simulink model "Palak_Plant_V1"  (R2025a)
settings: Solver=VariableStepAuto  StartTime=0.0  StopTime=10.0  RelTol=1e-3
settings Model: Creator=palak  LastModifiedBy=palak

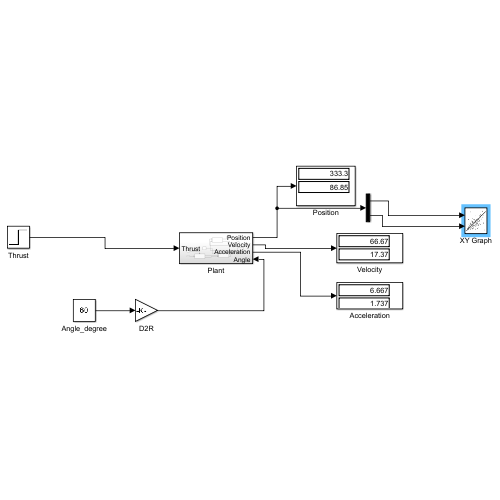
[thumbnail: Simulink's stored preview of the top-level diagram]
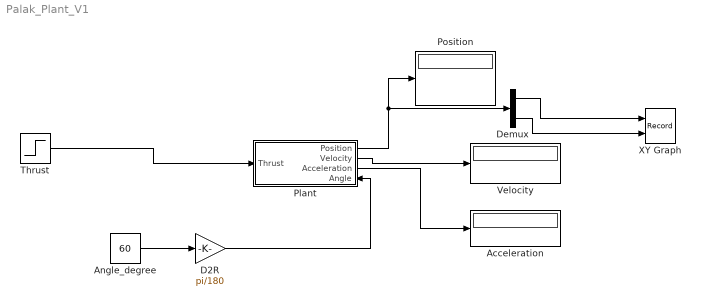
== system Palak_Plant_V1 ==
  Acceleration : Display
  Angle_degree : Constant  Value=60
  D2R : Gain  Gain=pi/180
  Demux : Demux  Outputs=2
  Plant : Subsystem
      settings: PortSchema="{\"entries\":[{\"content\":{\"sides\":[{\"content\":{\"connectorIds\":[\"In1\"]},\"type\":\"ConnectorPlacement.EquallySpacedRectSide\",\"uuid\":\"5de75d20-e3de-4891-9f30-3a0def6c848b\"},{\"content\":{\"connectorIds\":[\"Out1\",\"Out2\",\"Out3\",\"In2\"],\"side\":\"RIGHT\"},\"type\":\"ConnectorPlacement.EquallySpacedRectSide\",\"uuid\":\"db51dd8a-e2b5-4d79-9796-924119c6ed6f\"},{\"content\":{\"side\":\"TOP\"},\"type\":\"ConnectorPlacement.EquallySpacedRectSide\",\"uuid\":\"19ab0691-ef15-4f63-9283-6db2c82ddebe\"}]},\"type\":\"ConnectorPlacement.EquallySpacedConnector\",\"uuid\":\"28e9291f-ce5a-4baf-96c8-583588e41189\"}],\"packageUris\":[\"http://schema.mathworks.com/mf0/Connector/R2020b\"],\"version\":\"1.0\"}"
  Position : Display
  Thrust : Step  Time=0  After=200  SampleTime=0
  Velocity : Display
  XY Graph : Record  NumPorts=2.0  FileSettingsInternal="{\"entries\":[{\"content\":{\"excelSettings\":{\"content\":{},\"type\":\"Streamout.ExcelSettings\"},\"parquetSettings\":{\"content\":{},\"type\":\"Streamout.ParquetSettings\"}},\"type\":\"Streamout.FileSettingStorage\",\"uuid\":\"\"}],\"packageUris\":[\"http:\\/\\/schema.mathworks.com\\/mf0\\/streamout_blocks\\/R2020a\"],\"version\":\"1.0\"}"  FrameSettings=[0, 0]  Layout=[1 1]  SignalsInternal="{\"entries\":[{\"content\":{\"signals\":[{\"content\":{\"blockPath\":[],\"dimensions\":[1],\"domain\":\"\",\"lineColor\":\"#0072bd\",\"lineWidth\":2,\"plots\":[ 1 ],\"port\":1,\"sid\":[\"\"],\"signalID\":1,\"signalName\":\"Demux:1\"},\"type\":\"RecordBlkView.Signal\",\"uuid\":\"\"},{\"content\":{\"blockPath\":[],\"dimensions\":[1],\"domain\":\"\",\"lineColor\":\"#d95319\",\"lineWidth\":2,\"plots\":[ 1 ],\"port\":2,\"sid\":[\"\"],\"signalID\":2,\"signalName\":\"Demux:2\"},\"type\":\"RecordBlkView.Signal\",\"uuid\":\"\"}]},\"type\":\"RecordBlkView.InputSignals\",\"uuid\":\"\"}],\"packageUris\":[\"http:\\/\\/schema.mathworks.com\\/mf0\\/streamout_blocks\\/R2020a\"],\"version\":\"1.0\"}"  VisualizationBindings="{\"xyplotplugin\":{\"info\":[{\"series\":[{\"bindingParametersList\":[{\"parameter\":\"X-Axis\",\"signalID\":1,\"signalName\":\"Demux:1\"},{\"parameter\":\"Y-Axis\",\"signalID\":2,\"signalName\":\"Demux:2\"}],\"seriesID\":0}],\"subplotID\":1}]}}"  CompatibilityTag=XY  st=-1
  wires:
  Angle_degree/1 -> D2R/1
  Thrust/1 -> Plant/1(Thrust)
  D2R/1 -> Plant/2(Angle)
  Plant/1(Position) -> Demux/1, Position/1
  Plant/2(Velocity) -> Velocity/1
  Plant/3(Acceleration) -> Acceleration/1
  Demux/1 -> XY Graph/1
  Demux/2 -> XY Graph/2

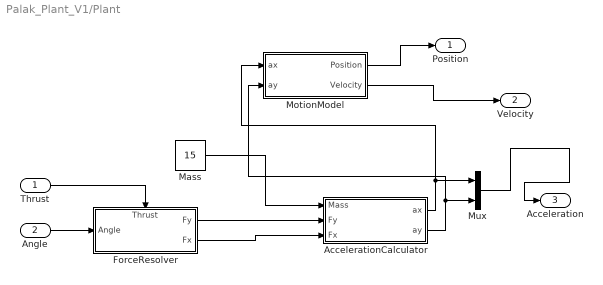
== system Palak_Plant_V1/Plant ==
  Thrust : Inport
  Angle : Inport  Port=2
  AccelerationCalculator : Subsystem
  ForceResolver : Subsystem
      settings: PortSchema="{\"entries\":[{\"content\":{\"sides\":[{\"content\":{\"connectorIds\":[\"In1\"]},\"type\":\"ConnectorPlacement.EquallySpacedRectSide\",\"uuid\":\"5de75d20-e3de-4891-9f30-3a0def6c848b\"},{\"content\":{\"connectorIds\":[\"Out1\",\"Out2\"],\"side\":\"RIGHT\"},\"type\":\"ConnectorPlacement.EquallySpacedRectSide\",\"uuid\":\"db51dd8a-e2b5-4d79-9796-924119c6ed6f\"},{\"content\":{\"connectorIds\":[\"In2\"],\"side\":\"TOP\"},\"type\":\"ConnectorPlacement.EquallySpacedRectSide\",\"uuid\":\"19ab0691-ef15-4f63-9283-6db2c82ddebe\"}]},\"type\":\"ConnectorPlacement.EquallySpacedConnector\",\"uuid\":\"28e9291f-ce5a-4baf-96c8-583588e41189\"}],\"packageUris\":[\"http://schema.mathworks.com/mf0/Connector/R2020b\"],\"version\":\"1.0\"}"
  Mass : Constant  Value=15
  MotionModel : Subsystem
  Mux : Mux  Inputs=2
  Position : Outport
  Velocity : Outport  Port=2
  Acceleration : Outport  Port=3
  wires:
  Angle/1 -> ForceResolver/1(Angle)
  Thrust/1 -> ForceResolver/2(Thrust)
  AccelerationCalculator/1(ax) -> MotionModel/1(ax), Mux/1
  Mass/1 -> AccelerationCalculator/1(Mass)
  ForceResolver/2(Fx) -> AccelerationCalculator/3(Fx)
  ForceResolver/1(Fy) -> AccelerationCalculator/2(Fy)
  AccelerationCalculator/2(ay) -> Mux/2, MotionModel/2(ay)
  Mux/1 -> Acceleration/1
  MotionModel/1(Position) -> Position/1
  MotionModel/2(Velocity) -> Velocity/1

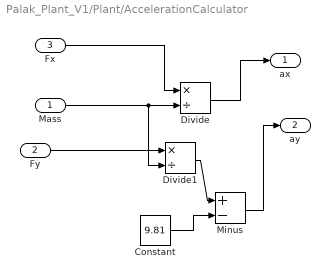
== system Palak_Plant_V1/Plant/AccelerationCalculator ==
  Mass : Inport
  Fy : Inport  Port=2
  Fx : Inport  Port=3
  Constant : Constant  Value=9.81
  Divide : Product  Inputs=*/
  Divide1 : Product  Inputs=*/
  Minus : Sum  Inputs=+-
  ax : Outport
  ay : Outport  Port=2
  wires:
  Mass/1 -> Divide1/2, Divide/2
  Fx/1 -> Divide/1
  Fy/1 -> Divide1/1
  Divide/1 -> ax/1
  Divide1/1 -> Minus/1
  Constant/1 -> Minus/2
  Minus/1 -> ay/1

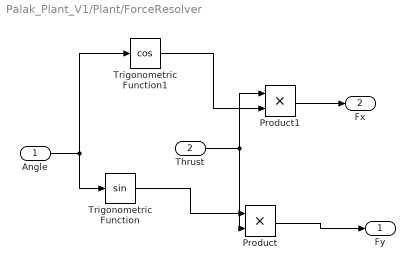
== system Palak_Plant_V1/Plant/ForceResolver ==
  Angle : Inport
  Thrust : Inport  Port=2
  Product : Product
  Product1 : Product
  Trigonometric Function : Trigonometry
  Trigonometric Function1 : Trigonometry  Operator=cos
  Fy : Outport
  Fx : Outport  Port=2
  wires:
  Angle/1 -> Trigonometric Function1/1, Trigonometric Function/1
  Trigonometric Function1/1 -> Product1/2
  Product1/1 -> Fx/1
  Trigonometric Function/1 -> Product/1
  Thrust/1 -> Product1/1, Product/2
  Product/1 -> Fy/1

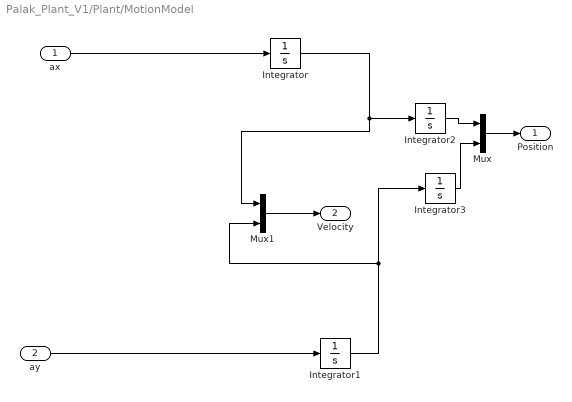
== system Palak_Plant_V1/Plant/MotionModel ==
  ax : Inport
  ay : Inport  Port=2
  Integrator{,1..3} (4 alike) : Integrator
  Mux : Mux  Inputs=2
  Mux1 : Mux  Inputs=2
  Position : Outport
  Velocity : Outport  Port=2
  wires:
  ax/1 -> Integrator/1
  ay/1 -> Integrator1/1
  Integrator/1 -> Mux1/1, Integrator2/1
  Integrator2/1 -> Mux/1
  Integrator1/1 -> Integrator3/1, Mux1/2
  Integrator3/1 -> Mux/2
  Mux/1 -> Position/1
  Mux1/1 -> Velocity/1
